simulink model "SR_Stage1"  (R2024b)
settings: Solver=ode4  StartTime=0.0  StopTime=P.Tend  FixedStep=P.Ts  RelTol=1e-3
InitFcn:
  | sr_params; TR = sr_track(P, trackType);
undefined symbols (not defined in the file): P, TR
settings Model: Creator=sange  LastModifiedBy=sange
settings DataIOCC: SaveOutput=off

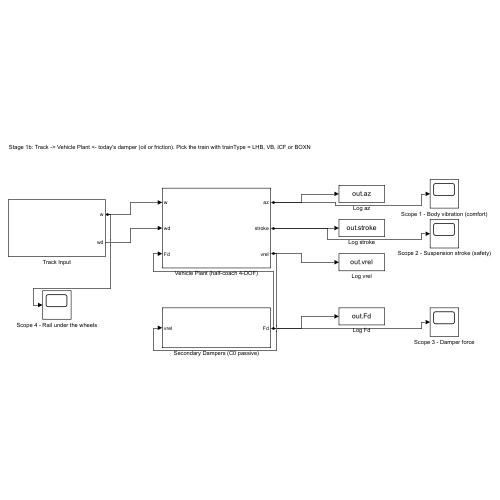
[thumbnail: Simulink's stored preview of the top-level diagram]
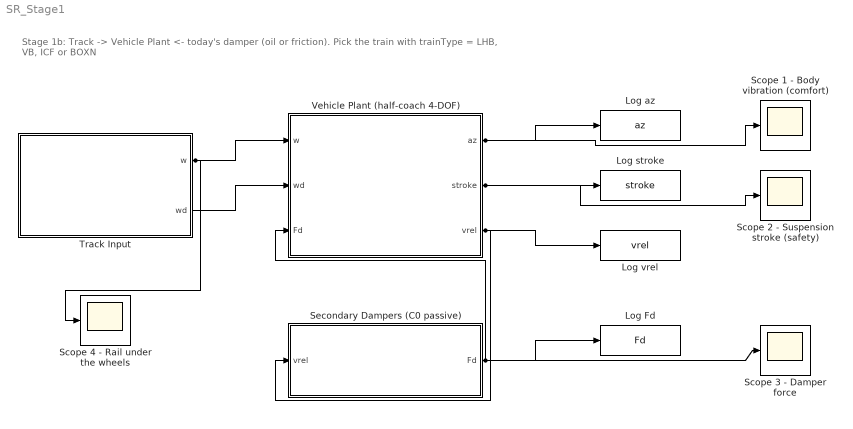
== system SR_Stage1 ==
  note: Stage 1b: Track -> Vehicle Plant <- today's damper (oil or friction). Pick the train with trainType = LHB, VB, ICF or BOXN
  Log Fd : ToWorkspace  VariableName=Fd  SaveFormat=Timeseries  SampleTime=-1
  Log az : ToWorkspace  VariableName=az  SaveFormat=Timeseries  SampleTime=-1
  Log stroke : ToWorkspace  VariableName=stroke  SaveFormat=Timeseries  SampleTime=-1
  Log vrel : ToWorkspace  VariableName=vrel  SaveFormat=Timeseries  SampleTime=-1
  Scope 1 - Body vibration (comfort) : Scope
  Scope 2 - Suspension stroke (safety) : Scope
  Scope 3 - Damper force : Scope
  Scope 4 - Rail under the wheels : Scope
  Secondary Dampers (C0 passive) : Subsystem  Description=Today's damping. Coaches: oil damper, force = c_s x stroke velocity. Casnub goods bogie: friction wedges, force = mu x load (smoothed). Replaced by the smart damper in Stage 2.
  Track Input : Subsystem  Description=Generates the vertical rail irregularity under each of the 4 wheels. Each wheel sees the same rail, delayed by its distance behind the lead wheel.
  Vehicle Plant (half-coach 4-DOF) : Subsystem  Description=Coach body (bounce + pitch) on two bogies. Secondary suspension = air spring (inside the equations) + damper force Fd (input). Primary suspension = springs + dampers to 4 wheelsets.
  wires:
  Track Input/1(w) -> Vehicle Plant (half-coach 4-DOF)/1(w), Scope 4 - Rail under the wheels/1
  Track Input/2(wd) -> Vehicle Plant (half-coach 4-DOF)/2(wd)
  Secondary Dampers (C0 passive)/1(Fd) -> Vehicle Plant (half-coach 4-DOF)/3(Fd), Log Fd/1, Scope 3 - Damper force/1
  Vehicle Plant (half-coach 4-DOF)/3(vrel) -> Secondary Dampers (C0 passive)/1(vrel), Log vrel/1
  Vehicle Plant (half-coach 4-DOF)/1(az) -> Log az/1, Scope 1 - Body vibration (comfort)/1
  Vehicle Plant (half-coach 4-DOF)/2(stroke) -> Log stroke/1, Scope 2 - Suspension stroke (safety)/1

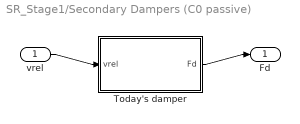
== system SR_Stage1/Secondary Dampers (C0 passive) ==
  vrel : Inport
  Today's damper : MATLAB Function  TreatAsAtomicUnit=on
  Fd : Outport
  wires:
  vrel/1 -> Today's damper/1(vrel)
  Today's damper/1(Fd) -> Fd/1

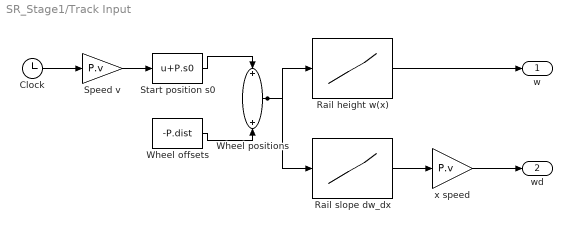
== system SR_Stage1/Track Input ==
  Clock : Clock
  Rail height w(x) : Lookup_n-D  NumberOfTableDimensions=1  BreakpointsForDimension1=TR.x  Table=TR.w  ExtrapMethod=Clip  InternalRulePriority=Speed  RndMeth=Simplest
  Rail slope dw_dx : Lookup_n-D  NumberOfTableDimensions=1  BreakpointsForDimension1=TR.x  Table=TR.dwdx  ExtrapMethod=Clip  InternalRulePriority=Speed  RndMeth=Simplest
  Speed v : Gain  Gain=P.v
  Start position s0 : Bias  Bias=P.s0  SaturateOnIntegerOverflow=off
  Wheel offsets : Constant  Value=-P.dist
  Wheel positions : Sum
  x speed : Gain  Gain=P.v
  w : Outport
  wd : Outport  Port=2
  wires:
  Clock/1 -> Speed v/1
  Speed v/1 -> Start position s0/1
  Start position s0/1 -> Wheel positions/1
  Wheel offsets/1 -> Wheel positions/2
  Wheel positions/1 -> Rail height w(x)/1, Rail slope dw_dx/1
  Rail height w(x)/1 -> w/1
  Rail slope dw_dx/1 -> x speed/1
  x speed/1 -> wd/1

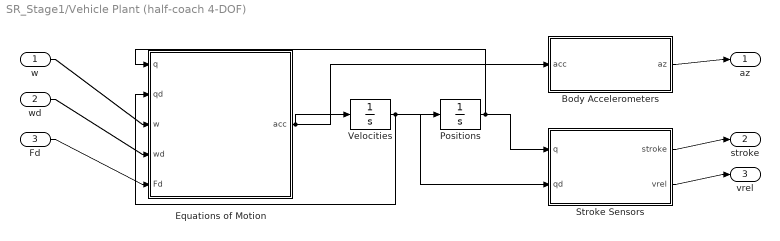
== system SR_Stage1/Vehicle Plant (half-coach 4-DOF) ==
  w : Inport
  wd : Inport  Port=2
  Fd : Inport  Port=3
  Body Accelerometers : MATLAB Function  TreatAsAtomicUnit=on
  Equations of Motion : MATLAB Function  TreatAsAtomicUnit=on
  Positions : Integrator  InitialCondition=zeros(4,1)
  Stroke Sensors : MATLAB Function  TreatAsAtomicUnit=on
  Velocities : Integrator  InitialCondition=zeros(4,1)
  az : Outport
  stroke : Outport  Port=2
  vrel : Outport  Port=3
  wires:
  Positions/1 -> Equations of Motion/1(q), Stroke Sensors/1(q)
  Velocities/1 -> Equations of Motion/2(qd), Positions/1, Stroke Sensors/2(qd)
  w/1 -> Equations of Motion/3(w)
  wd/1 -> Equations of Motion/4(wd)
  Fd/1 -> Equations of Motion/5(Fd)
  Equations of Motion/1(acc) -> Velocities/1, Body Accelerometers/1(acc)
  Body Accelerometers/1(az) -> az/1
  Stroke Sensors/1(stroke) -> stroke/1
  Stroke Sensors/2(vrel) -> vrel/1

== matlab function SR_Stage1/Vehicle Plant (half-coach 4-DOF)/Body Accelerometers ==
  data: acc input; az output size=[3 1]; P parameter
function az = fcn(acc, P)
% Body acceleration at the centre and above each bogie (comfort).
az = sr_measure(zeros(4,1), zeros(4,1), acc, P);

== matlab function SR_Stage1/Vehicle Plant (half-coach 4-DOF)/Equations of Motion ==
  data: q input; acc output size=[4 1]; qd input; w input; wd input; Fd input; P parameter
function acc = fcn(q, qd, w, wd, Fd, P)
% Newton's law for body bounce, body pitch and the two bogie frames.
acc = sr_eom(q, qd, w, wd, Fd, P);

== matlab function SR_Stage1/Vehicle Plant (half-coach 4-DOF)/Stroke Sensors ==
  data: q input; stroke output size=[2 1]; qd input; vrel output size=[2 1]; P parameter
function [stroke, vrel] = fcn(q, qd, P)
% Suspension stroke (safety) and stroke velocity (what the damper feels).
[~, stroke, vrel] = sr_measure(q, qd, zeros(4,1), P);

== matlab function SR_Stage1/Secondary Dampers (C0 passive)/Today's damper ==
  data: vrel input; Fd output size=[2 1]; P parameter
function Fd = fcn(vrel, P)
% Oil damper (viscous, c_s) + friction wedges (Casnub, F_fr). One of the two is zero.
Fd = P.cs * vrel + P.Ffr * tanh(vrel / P.veps);
